simulink model "drone_windshear_pid"  (R2019a)
settings: Solver=ode45  StartTime=0.0  StopTime=tstop  MaxStep=0.01  RelTol=1e-3
values from neighbouring files (symbols this model uses):
  alphas = 0.2    [drone_windshear_params.m]
  Aw = 3    [drone_windshear_params.m]
  cdx = 0.30    (= 0.3)    [drone_windshear_params.m]
  cdz = 0.40    (= 0.4)    [drone_windshear_params.m]
  g = 9.81    [drone_windshear_params.m]
  J = 0.03    [drone_windshear_params.m]
  kq = 0.02    [drone_windshear_params.m]
  m = 1.5    [drone_windshear_params.m]
  ShearOn = 1    [drone_windshear_params.m]
  t0 = 10    [drone_windshear_params.m]
  tau_m = 0.03    [drone_windshear_params.m]
  taumax = 1.5    [drone_windshear_params.m]
  th_Kd = 0.63    [drone_windshear_params.m]
  th_Ki = 0.0    (= 0)    [drone_windshear_params.m]
  th_Kp = 6.75    [drone_windshear_params.m]
  th_N = 40    [drone_windshear_params.m]
  theta_max = deg2rad(25)    [drone_windshear_params.m]
  Tshear = 8    [drone_windshear_params.m]
  Ug = 8    [drone_windshear_params.m]
  x_Kd = 0.245    [drone_windshear_params.m]
  x_Ki = 0.03    [drone_windshear_params.m]
  x_Kp = 0.23    [drone_windshear_params.m]
  x_N = 10    [drone_windshear_params.m]
  xcmd = 0    [drone_windshear_params.m]
  z0 = 30    [drone_windshear_params.m]
  z_Kd = 7.2    [drone_windshear_params.m]
  z_Ki = 5.0    (= 5)    [drone_windshear_params.m]
  z_Kp = 13.5    [drone_windshear_params.m]
  z_N = 20    [drone_windshear_params.m]
  zcmd = 0    [drone_windshear_params.m]
libraries: simulink x3
settings Model: Creator=ABHI  LastModifiedBy=ABHI

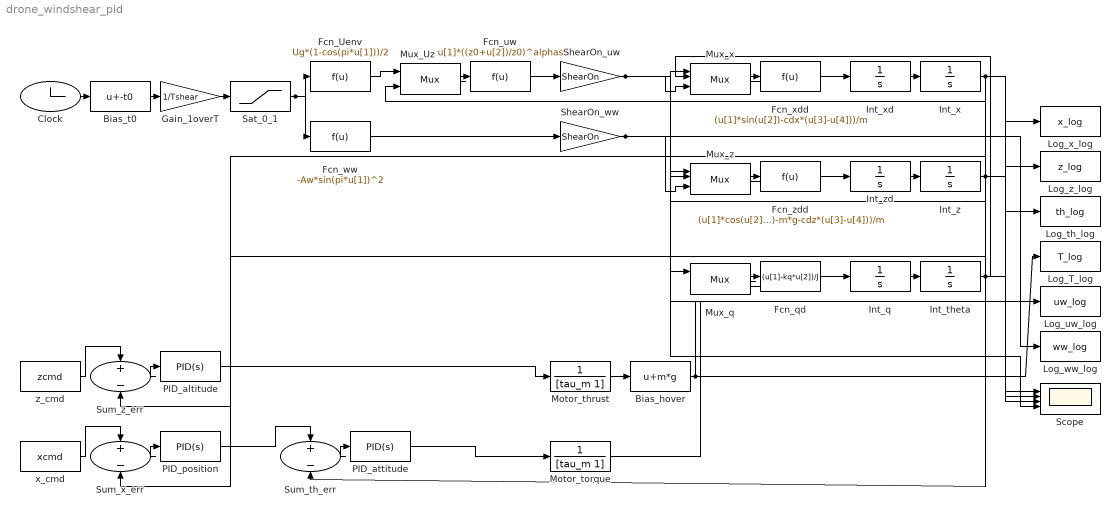
== system drone_windshear_pid ==
  Bias_hover : Bias  Bias=m*g
  Bias_t0 : Bias  Bias=-t0
  Clock : Clock
  Fcn_Uenv : Fcn  Expr=Ug*(1-cos(pi*u[1]))/2
  Fcn_qd : Fcn  Expr=(u[1]-kq*u[2])/J
  Fcn_uw : Fcn  Expr=u[1]*((z0+u[2])/z0)^alphas
  Fcn_ww : Fcn  Expr=-Aw*sin(pi*u[1])^2
  Fcn_xdd : Fcn  Expr=(u[1]*sin(u[2])-cdx*(u[3]-u[4]))/m
  Fcn_zdd : Fcn  Expr=(u[1]*cos(u[2])-m*g-cdz*(u[3]-u[4]))/m
  Gain_1overT : Gain  Gain=1/Tshear
  Int_q : Integrator
  Int_theta : Integrator
  Int_x : Integrator
  Int_xd : Integrator
  Int_z : Integrator
  Int_zd : Integrator
  Log_T_log : ToWorkspace  VariableName=T_log  SaveFormat=Timeseries  SampleTime=-1
  Log_th_log : ToWorkspace  VariableName=th_log  SaveFormat=Timeseries  SampleTime=-1
  Log_uw_log : ToWorkspace  VariableName=uw_log  SaveFormat=Timeseries  SampleTime=-1
  Log_ww_log : ToWorkspace  VariableName=ww_log  SaveFormat=Timeseries  SampleTime=-1
  Log_x_log : ToWorkspace  VariableName=x_log  SaveFormat=Timeseries  SampleTime=-1
  Log_z_log : ToWorkspace  VariableName=z_log  SaveFormat=Timeseries  SampleTime=-1
  Motor_thrust : TransferFcn  Numerator=1  Denominator=[tau_m 1]
  Motor_torque : TransferFcn  Numerator=1  Denominator=[tau_m 1]
  Mux_Uz : Mux  Inputs=2
  Mux_q : Mux  Inputs=2
  Mux_x : Mux
  Mux_z : Mux
  PID_altitude : simulink/Continuous/PID Controller  Controller=PID  Form=Parallel  TimeDomain=Continuous-time  SampleTime=-1  IntegratorMethod=Forward Euler  FilterMethod=Forward Euler  ControllerParametersSource=internal  P=z_Kp  I=z_Ki  D=z_Kd  UseFilter=on  N=z_N  TunerSelectOption=Transfer Function Based (PID Tuner App)  InitialConditionSource=internal  InitialConditionForIntegrator=0  InitialConditionForFilter=0  DifferentiatorICPrevScaledInput=0  ExternalReset=none  TrackingMode=off  Kt=1  LimitOutput=on  UpperSaturationLimit=m*g  LowerSaturationLimit=-m*g  LinearizeAsGain=on  AntiWindupMode=clamping  Kb=1  POutMin=[]  POutMax=[]  IOutMin=[]  IOutMax=[]  DOutMin=[]  DOutMax=[]  NOutMin=[]  NOutMax=[]  SumOutMin=[]  SumOutMax=[]  SaturationOutMin=[]  SaturationOutMax=[]  PParamMin=[]  PParamMax=[]  IParamMin=[]  IParamMax=[]  DParamMin=[]  DParamMax=[]  NParamMin=[]  NParamMax=[]  KbParamMin=[]  KbParamMax=[]  KtParamMin=[]  KtParamMax=[]  KbOutMin=[]  KbOutMax=[]  KtOutMin=[]  KtOutMax=[]  IntegratorOutMin=[]  IntegratorOutMax=[]  FilterOutMin=[]  FilterOutMax=[]  SumI1OutMin=[]  SumI1OutMax=[]  SumI2OutMin=[]  SumI2OutMax=[]  SumI3OutMin=[]  SumI3OutMax=[]  SumI4OutMin=[]  SumI4OutMax=[]  SumDOutMin=[]  SumDOutMax=[]  DifferentiatorOutMin=[]  DifferentiatorOutMax=[]  FilterDiffOutCoefMin=[]  FilterDiffOutCoefMax=[]  ReciprocalOutMin=[]  ReciprocalOutMax=[]  SumDenOutMin=[]  SumDenOutMax=[]  SumNumOutMin=[]  SumNumOutMax=[]  DivideOutMin=[]  DivideOutMax=[]  IntegratorContinuousStateAttributes=''  IntegratorStateMustResolveToSignalObject=off  IntegratorRTWStateStorageClass=Auto  FilterContinuousStateAttributes=''  FilterStateMustResolveToSignalObject=off  FilterRTWStateStorageClass=Auto  ParallelPVariant=InternalParameters  IdealPVariant=Disabled  IVariant=InternalParameters  DVariant=InternalParameters  IntegratorVariant=Continuous  SatVariant=Enabled  AWVariant=ContClampingParallel  PCopyVariant=Disabled  TRVariant=Disabled  FdbkBlocksVariant=Forward  IdealPFdbkVariant=Disabled  SatFdbkVariant=Disabled  DerivativeFilterVariant=ContFilter  NVariant=InternalParameters  NCopyVariant=Disabled  FilterICVariant=InternalICsFilter  IntegratorICVariant=InternalICs  ExternalResetVariant=Disabled  TRSumVariant=Passthrough  SumFdbkVariant=Disabled  SumVariant=Sum_PID
  PID_attitude : simulink/Continuous/PID Controller  Controller=PID  Form=Parallel  TimeDomain=Continuous-time  SampleTime=-1  IntegratorMethod=Forward Euler  FilterMethod=Forward Euler  ControllerParametersSource=internal  P=th_Kp  I=th_Ki  D=th_Kd  UseFilter=on  N=th_N  TunerSelectOption=Transfer Function Based (PID Tuner App)  InitialConditionSource=internal  InitialConditionForIntegrator=0  InitialConditionForFilter=0  DifferentiatorICPrevScaledInput=0  ExternalReset=none  TrackingMode=off  Kt=1  LimitOutput=on  UpperSaturationLimit=taumax  LowerSaturationLimit=-taumax  LinearizeAsGain=on  AntiWindupMode=clamping  Kb=1  POutMin=[]  POutMax=[]  IOutMin=[]  IOutMax=[]  DOutMin=[]  DOutMax=[]  NOutMin=[]  NOutMax=[]  SumOutMin=[]  SumOutMax=[]  SaturationOutMin=[]  SaturationOutMax=[]  PParamMin=[]  PParamMax=[]  IParamMin=[]  IParamMax=[]  DParamMin=[]  DParamMax=[]  NParamMin=[]  NParamMax=[]  KbParamMin=[]  KbParamMax=[]  KtParamMin=[]  KtParamMax=[]  KbOutMin=[]  KbOutMax=[]  KtOutMin=[]  KtOutMax=[]  IntegratorOutMin=[]  IntegratorOutMax=[]  FilterOutMin=[]  FilterOutMax=[]  SumI1OutMin=[]  SumI1OutMax=[]  SumI2OutMin=[]  SumI2OutMax=[]  SumI3OutMin=[]  SumI3OutMax=[]  SumI4OutMin=[]  SumI4OutMax=[]  SumDOutMin=[]  SumDOutMax=[]  DifferentiatorOutMin=[]  DifferentiatorOutMax=[]  FilterDiffOutCoefMin=[]  FilterDiffOutCoefMax=[]  ReciprocalOutMin=[]  ReciprocalOutMax=[]  SumDenOutMin=[]  SumDenOutMax=[]  SumNumOutMin=[]  SumNumOutMax=[]  DivideOutMin=[]  DivideOutMax=[]  IntegratorContinuousStateAttributes=''  IntegratorStateMustResolveToSignalObject=off  IntegratorRTWStateStorageClass=Auto  FilterContinuousStateAttributes=''  FilterStateMustResolveToSignalObject=off  FilterRTWStateStorageClass=Auto  ParallelPVariant=InternalParameters  IdealPVariant=Disabled  IVariant=InternalParameters  DVariant=InternalParameters  IntegratorVariant=Continuous  SatVariant=Enabled  AWVariant=ContClampingParallel  PCopyVariant=Disabled  TRVariant=Disabled  FdbkBlocksVariant=Forward  IdealPFdbkVariant=Disabled  SatFdbkVariant=Disabled  DerivativeFilterVariant=ContFilter  NVariant=InternalParameters  NCopyVariant=Disabled  FilterICVariant=InternalICsFilter  IntegratorICVariant=InternalICs  ExternalResetVariant=Disabled  TRSumVariant=Passthrough  SumFdbkVariant=Disabled  SumVariant=Sum_PID
  PID_position : simulink/Continuous/PID Controller  Controller=PID  Form=Parallel  TimeDomain=Continuous-time  SampleTime=-1  IntegratorMethod=Forward Euler  FilterMethod=Forward Euler  ControllerParametersSource=internal  P=x_Kp  I=x_Ki  D=x_Kd  UseFilter=on  N=x_N  TunerSelectOption=Transfer Function Based (PID Tuner App)  InitialConditionSource=internal  InitialConditionForIntegrator=0  InitialConditionForFilter=0  DifferentiatorICPrevScaledInput=0  ExternalReset=none  TrackingMode=off  Kt=1  LimitOutput=on  UpperSaturationLimit=theta_max  LowerSaturationLimit=-theta_max  LinearizeAsGain=on  AntiWindupMode=clamping  Kb=1  POutMin=[]  POutMax=[]  IOutMin=[]  IOutMax=[]  DOutMin=[]  DOutMax=[]  NOutMin=[]  NOutMax=[]  SumOutMin=[]  SumOutMax=[]  SaturationOutMin=[]  SaturationOutMax=[]  PParamMin=[]  PParamMax=[]  IParamMin=[]  IParamMax=[]  DParamMin=[]  DParamMax=[]  NParamMin=[]  NParamMax=[]  KbParamMin=[]  KbParamMax=[]  KtParamMin=[]  KtParamMax=[]  KbOutMin=[]  KbOutMax=[]  KtOutMin=[]  KtOutMax=[]  IntegratorOutMin=[]  IntegratorOutMax=[]  FilterOutMin=[]  FilterOutMax=[]  SumI1OutMin=[]  SumI1OutMax=[]  SumI2OutMin=[]  SumI2OutMax=[]  SumI3OutMin=[]  SumI3OutMax=[]  SumI4OutMin=[]  SumI4OutMax=[]  SumDOutMin=[]  SumDOutMax=[]  DifferentiatorOutMin=[]  DifferentiatorOutMax=[]  FilterDiffOutCoefMin=[]  FilterDiffOutCoefMax=[]  ReciprocalOutMin=[]  ReciprocalOutMax=[]  SumDenOutMin=[]  SumDenOutMax=[]  SumNumOutMin=[]  SumNumOutMax=[]  DivideOutMin=[]  DivideOutMax=[]  IntegratorContinuousStateAttributes=''  IntegratorStateMustResolveToSignalObject=off  IntegratorRTWStateStorageClass=Auto  FilterContinuousStateAttributes=''  FilterStateMustResolveToSignalObject=off  FilterRTWStateStorageClass=Auto  ParallelPVariant=InternalParameters  IdealPVariant=Disabled  IVariant=InternalParameters  DVariant=InternalParameters  IntegratorVariant=Continuous  SatVariant=Enabled  AWVariant=ContClampingParallel  PCopyVariant=Disabled  TRVariant=Disabled  FdbkBlocksVariant=Forward  IdealPFdbkVariant=Disabled  SatFdbkVariant=Disabled  DerivativeFilterVariant=ContFilter  NVariant=InternalParameters  NCopyVariant=Disabled  FilterICVariant=InternalICsFilter  IntegratorICVariant=InternalICs  ExternalResetVariant=Disabled  TRSumVariant=Passthrough  SumFdbkVariant=Disabled  SumVariant=Sum_PID
  Sat_0_1 : Saturate  UpperLimit=1  LowerLimit=0
  Scope : Scope  NumInputPorts=4
  ShearOn_uw : Gain  Gain=ShearOn
  ShearOn_ww : Gain  Gain=ShearOn
  Sum_th_err : Sum  Inputs=+-
  Sum_x_err : Sum  Inputs=+-
  Sum_z_err : Sum  Inputs=+-
  x_cmd : Constant  Value=xcmd
  z_cmd : Constant  Value=zcmd
  wires:
  Clock/1 -> Bias_t0/1
  Bias_t0/1 -> Gain_1overT/1
  Gain_1overT/1 -> Sat_0_1/1
  Sat_0_1/1 -> Fcn_Uenv/1, Fcn_ww/1
  Fcn_Uenv/1 -> Mux_Uz/1
  Mux_Uz/1 -> Fcn_uw/1
  Fcn_uw/1 -> ShearOn_uw/1
  Fcn_ww/1 -> ShearOn_ww/1
  Mux_x/1 -> Fcn_xdd/1
  Fcn_xdd/1 -> Int_xd/1
  Int_xd/1 -> Int_x/1, Mux_x/3
  ShearOn_uw/1 -> Mux_x/4, Log_uw_log/1, Scope/4
  Mux_z/1 -> Fcn_zdd/1
  Fcn_zdd/1 -> Int_zd/1
  Int_zd/1 -> Int_z/1, Mux_z/3
  ShearOn_ww/1 -> Mux_z/4, Log_ww_log/1
  Mux_q/1 -> Fcn_qd/1
  Fcn_qd/1 -> Int_q/1
  Int_q/1 -> Int_theta/1, Mux_q/2
  Int_theta/1 -> Mux_x/2, Mux_z/2, Sum_th_err/2, Log_th_log/1, Scope/3
  Int_z/1 -> Mux_Uz/2, Sum_z_err/2, Log_z_log/1, Scope/2
  Motor_thrust/1 -> Bias_hover/1
  Bias_hover/1 -> Mux_x/1, Mux_z/1, Log_T_log/1
  Motor_torque/1 -> Mux_q/1
  z_cmd/1 -> Sum_z_err/1
  Sum_z_err/1 -> PID_altitude/1
  PID_altitude/1 -> Motor_thrust/1
  x_cmd/1 -> Sum_x_err/1
  Int_x/1 -> Sum_x_err/2, Log_x_log/1, Scope/1
  Sum_x_err/1 -> PID_position/1
  PID_position/1 -> Sum_th_err/1
  Sum_th_err/1 -> PID_attitude/1
  PID_attitude/1 -> Motor_torque/1
